simulink model "experiment_supervisor_user"  (R2025b)
settings: Solver=FixedStepDiscrete  StartTime=0.0  StopTime=inf  RelTol=1e-3
PreLoadFcn:
  | run('experiment_supervisor_data');
model workspace (MAT data in the model file):
  Ts = 0.01
undefined symbols (not defined in the file or in its folder): ControlModes, ind, MCControlModes, MCMotorParamsSet
libraries: dspswit3 x1, sldrtlib x1
settings Model: DataDictionary=amcbldc.sldd  SimulationMode=accelerator  Creator=mfussi  LastModifiedBy=rpumpo
settings OptimizationCC: GainParamInheritBuiltInType=on  DefaultUnderspecifiedDataType=single  ReuseModelBlockBuffer=off  SimCompilerOptimization=on
settings DebuggingCC: ParamSuppressDoubleToSinglePrecisionLossMsg=on  UnconnectedInputMsg=warning  UnconnectedOutputMsg=warning  UnconnectedLineMsg=warning
settings HardwareCC: ProdBitPerLong=64.0  ProdHWDeviceType=Intel->x86-64 (Linux 64)
settings ModelReferenceCC: UpdateModelReferenceTargets=IfOutOfDate  EnableRefExpFcnMdlSchedulingChecks=on
settings RTWCC: SystemTargetFile=sldrt.tlc  TemplateMakefile=sldrt.tmf  TargetLang=C++  RTWCompilerOptimization=on  GPUComputeCapability=3.5  DLArmComputeVersion=19.05  Description=Simulink Desktop Real-Time
settings CodeAppCC: MaxIdLength=95.0
settings SimulinkDesktopRealTimeCC: ExtModeTransport=0.0  ExtModeStaticAllocSize=1000000.0  TargetLibSuffix=_sldrt.a  TargetPreCompLibLocation=C:\Program Files\MATLAB\R2025b\toolbox\sldrt\lib\win64  TargetLangStandard=C++11 (ISO)  MultiwordLength=2048.0  DynamicStringBufferSize=256.0  ParMdlRefBuildCompliant=on  PreserveMATLABNamespacesInGeneratedCode=on  SubcomponentCodeInterfacePackaging=Reusable function  OptimizeReductions=on

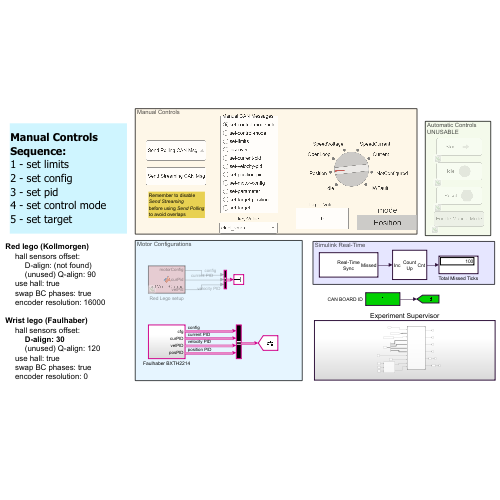
[thumbnail: Simulink's stored preview of the top-level diagram]
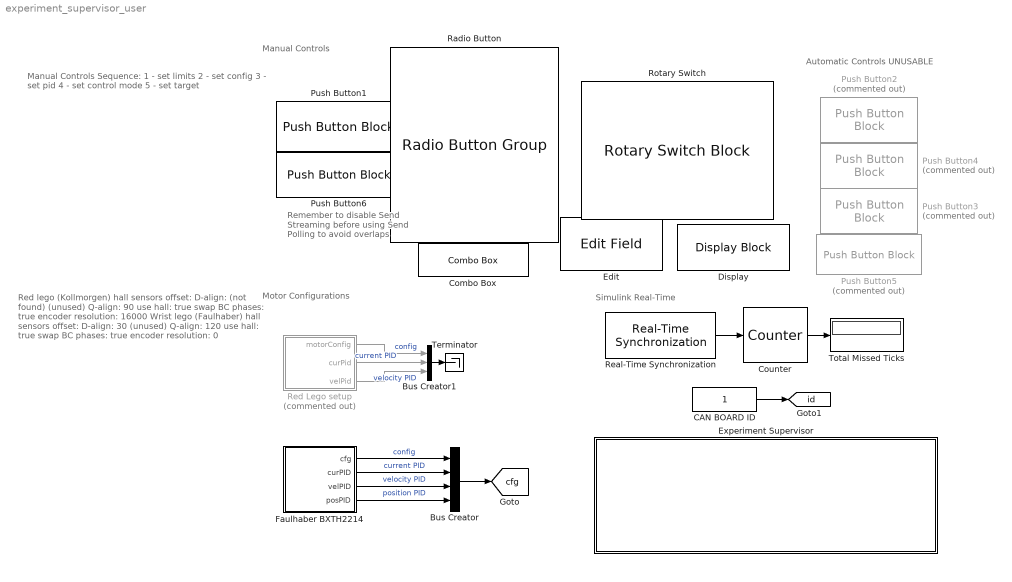
== system experiment_supervisor_user ==
  note: Manual Controls Sequence:
      | 1 - set limits
      | 2 - set config
      | 3 - set pid
      | 4 - set control mode
      | 5 - set target
  note: Motor Configurations
  note: Red lego (Kollmorgen)
      | hall sensors offset:
      | D-align: (not found)
      | (unused) Q-align: 90
      | use hall: true
      | swap BC phases: true
      | encoder resolution: 16000
      |
      | Wrist lego (Faulhaber)
      | hall sensors offset:
      | D-align: 30
      | (unused) Q-align: 120
      | use hall: true
      | swap BC phases: true
      | encoder resolution: 0
  note: Remember to disable
      | Send Streaming
      | before using Send Polling
      | to avoid overlaps
  note: Simulink Real-Time
  note: Manual Controls
  note: Automatic Controls
      | UNUSABLE
  Bus Creator : BusCreator  Inputs=4
  Bus Creator1 : BusCreator  Inputs=3
  CAN BOARD ID : Constant  OutDataTypeStr=uint32  SampleTime=0.01
  Combo Box : ComboBox  SelectedLabel=hall  UseEnumeratedDataType=on  EnumeratedDataType=MCMotorParamsSet
  Counter : dspswit3/Counter  Direction=Up  CountEvent=Rising edge  CounterSize=16 bits  MaxCount=10000  InitialCount=0  Output=Count  HitValue=32  ResetInput=off  SamplesPerFrame=1  Ts=1  CntDtype=uint16  HitDtype=Logical
  Display : DisplayBlock  Format=Integer  Transparency=1  GridColor=[0.502, 0.502, 0.502]
  Edit : EditField  ShowInitialText=on  Alignment=Center
  Experiment Supervisor : Subsystem
  Faulhaber BXTH2214 : Subsystem
  Push Button1 : PushButtonBlock  ButtonText=Send Polling CAN Msg  Icon=Triangle  IconAlignment=Right  IconOnColor=[1.0, 0.0, 1.0]  IconOffColor=[0.74901960784313726, 0.74901960784313726, 0.74901960784313726]  IconColor=On  OffValue=0.000000
  Push Button2 : PushButtonBlock  Commented=on  ButtonText=Start  Icon=TurnSignalRight  IconAlignment=Right  IconOnColor=[0.0, 1.0, 0.0]  IconOffColor=[0.74901960784313726, 0.74901960784313726, 0.74901960784313726]  IconColor=On  OffValue=-nan(ind)
  Push Button3 : PushButtonBlock  Commented=on  ButtonText=Reset  OnValue=2  Icon=Hexagon  IconAlignment=Right  IconOnColor=[1.0, 0.0, 0.0]  IconOffColor=[0.74901960784313726, 0.74901960784313726, 0.74901960784313726]  IconColor=On  OffValue=2.000000
  Push Button4 : PushButtonBlock  Commented=on  ButtonText=Idle  OnValue=0  Icon=Circle  IconAlignment=Right  IconOnColor=[1.0, 1.0, 0.0]  IconOffColor=[0.74901960784313726, 0.74901960784313726, 0.74901960784313726]  IconColor=On  OffValue=-1.000000
  Push Button5 : PushButtonBlock  Commented=on  ButtonText=Enable Manual Mode  ButtonType=Latch  IconAlignment=Right  IconOnColor=[1.0, 0.0, 1.0]  IconOffColor=[0.74901960784313726, 0.74901960784313726, 0.74901960784313726]  OffValue=0.000000
  Push Button6 : PushButtonBlock  ButtonText=Send Streaming CAN Msg  ButtonType=Latch  Icon=TurnSignalRight  IconAlignment=Right  IconOnColor=[0.0, 0.0, 1.0]  IconOffColor=[0.74901960784313726, 0.74901960784313726, 0.74901960784313726]  IconColor=On  OffValue=0.000000
  Radio Button : RadioButtonGroup  LabelPosition=Hide  SelectedLabel=set-control-mode-idle  ButtonGroupName=Manual CAN Messages
  Real-Time Synchronization : sldrtlib/Real-Time Synchronization  SampleTime=Ts  MaxMissedTicks=inf  ShowMissedTicks=on  YieldWhenWaiting=off
  Red Lego setup : MATLAB Function  Commented=on  TreatAsAtomicUnit=on
  Rotary Switch : RotarySwitchBlock  LabelPosition=Hide  UseEnumeratedDataType=on  EnumeratedDataType=MCControlModes
  Terminator : Terminator
  Total Missed Ticks : Display
      settings: Decimation=5
  tag scope: cfg=global, id=global
  wires:
  Real-Time Synchronization/1 -> Counter/1
  Faulhaber BXTH2214/1(cfg) -> Bus Creator/1  "config"
  Faulhaber BXTH2214/2(curPID) -> Bus Creator/2  "current PID"
  Faulhaber BXTH2214/3(velPID) -> Bus Creator/3  "velocity PID"
  Red Lego setup/3(velPid) -> Bus Creator1/3  "velocity PID"
  Red Lego setup/1(motorConfig) -> Bus Creator1/1  "config"
  Red Lego setup/2(curPid) -> Bus Creator1/2  "current PID"
  Bus Creator/1 -> [cfg]
  Bus Creator1/1 -> Terminator/1
  Counter/1 -> Total Missed Ticks/1
  CAN BOARD ID/1 -> [id]
  Faulhaber BXTH2214/4(posPID) -> Bus Creator/4  "position PID"

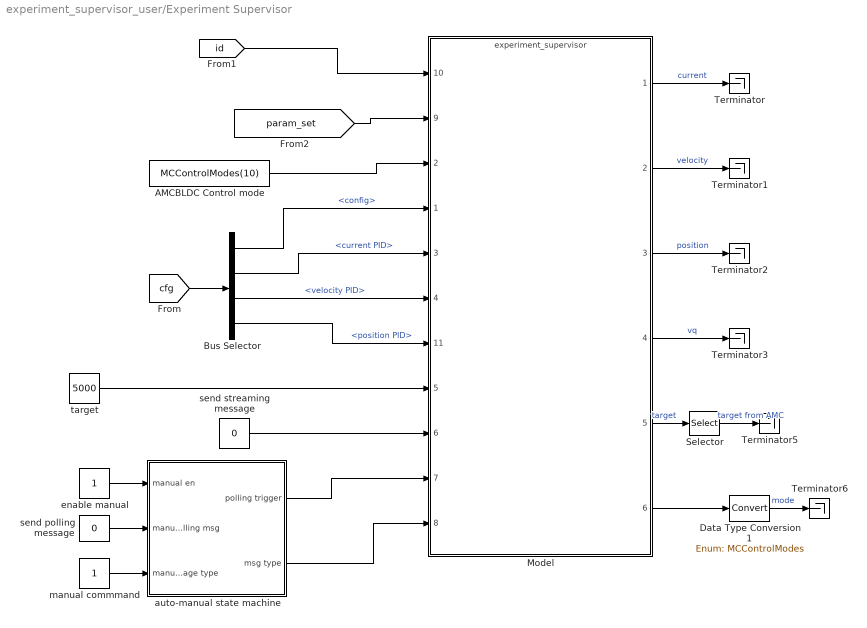
== system experiment_supervisor_user/Experiment Supervisor ==
  AMCBLDC Control mode : Constant  Value=MCControlModes(10)
  Bus Selector : BusSelector  OutputSignals=config,current PID,velocity PID,position PID
  Data Type Conversion1 : DataTypeConversion  OutDataTypeStr=Enum: MCControlModes  SaturateOnIntegerOverflow=off  RndMeth=Floor
  Model : ModelReference  ModelNameDialog=experiment_supervisor.slx  SimulationMode=Normal  ModelReferenceVersion=9.47
      settings: PortSchema="{\"entries\":[{\"content\":{\"sides\":[{\"content\":{\"connectorIds\":[\"In10\",\"In9\",\"In2\",\"In1\",\"In3\",\"In4\",\"In11\",\"In5\",\"In6\",\"In7\",\"In8\"]},\"type\":\"ConnectorPlacement.EquallySpacedRectSide\",\"uuid\":\"bfbdf898-42a5-495c-8a1e-d70d1f7414e8\"},{\"content\":{\"connectorIds\":[\"Out1\",\"Out2\",\"Out3\",\"Out4\",\"Out5\",\"Out6\"],\"side\":\"RIGHT\"},\"type\":\"ConnectorPlacement.EquallySpacedRectSide\",\"uuid\":\"3fb07422-e541-47fe-8bd2-34fc87b5d4e0\"},{\"content\":{\"side\":\"TOP\"},\"type\":\"ConnectorPlacement.EquallySpacedRectSide\",\"uuid\":\"cc070490-4dff-4736-882c-6ee4a91a824d\"}]},\"type\":\"ConnectorPlacement.EquallySpacedConnector\",\"uuid\":\"82f7e7bc-78f2-4fca-805f-7ff02feabc7a\"}],\"packageUris\":[\"http://schema.mathworks.com/mf0/Connector/R2020b\"],\"version\":\"1.0\"}"
  Selector : Selector  InputPortWidth=3  IndexOptions=Index vector (dialog)  Indices=[1]  OutputSizes=1
  Terminator{,1..3,5..6} (6 alike) : Terminator
  auto-manual state machine : Subsystem
  enable manual : Constant  OutDataTypeStr=uint8
  manual commmand : Constant  OutDataTypeStr=uint8
  send polling message : Constant  Value=0  OutDataTypeStr=uint8
  send streaming message : Constant  Value=0  OutDataTypeStr=Inherit: Inherit via back propagation
  target : Constant  Value=5000  OutDataTypeStr=single
  wires:
  Bus Selector/2 -> Model/3  "<current PID>"
  enable manual/1 -> auto-manual state machine/1(manual en)
  send polling message/1 -> auto-manual state machine/2(manual send polling msg)
  [cfg] -> Bus Selector/1
  Selector/1 -> Terminator5/1  "target from AMC"
  manual commmand/1 -> auto-manual state machine/3(manual message type)
  Model/3 -> Terminator2/1  "position"
  AMCBLDC Control mode/1 -> Model/2
  Bus Selector/1 -> Model/1  "<config>"
  Bus Selector/3 -> Model/4  "<velocity PID>"
  target/1 -> Model/5
  send streaming message/1 -> Model/6
  auto-manual state machine/1(polling trigger) -> Model/7
  Model/4 -> Terminator3/1  "vq"
  auto-manual state machine/2(msg type) -> Model/8
  Model/1 -> Terminator/1  "current"
  Model/2 -> Terminator1/1  "velocity"
  Model/5 -> Selector/1  "target"
  Model/6 -> Data Type Conversion1/1
  Data Type Conversion1/1 -> Terminator6/1  "mode"
  [id] -> Model/10
  [param_set] -> Model/9
  Bus Selector/4 -> Model/11  "<position PID>"

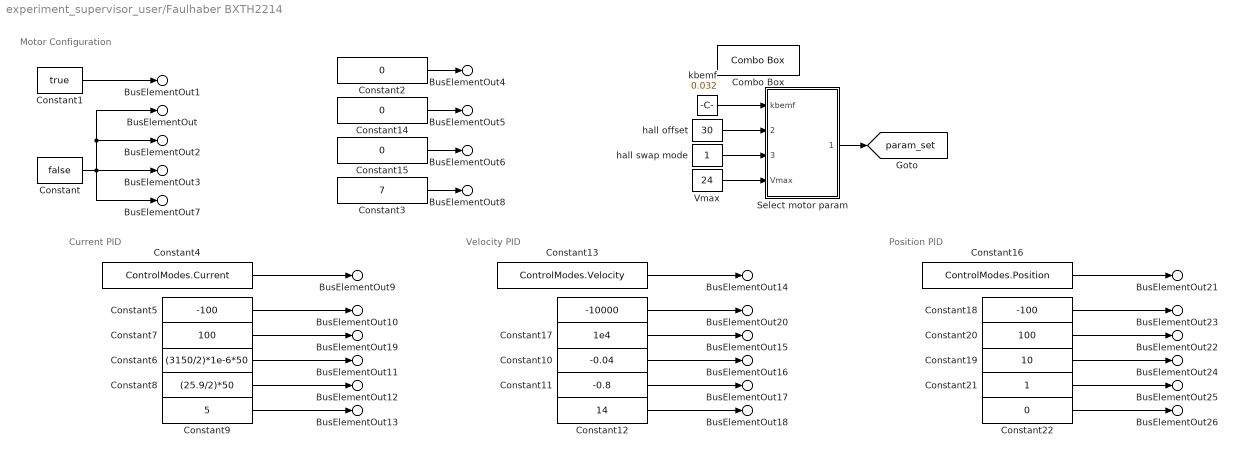
== system experiment_supervisor_user/Faulhaber BXTH2214 ==
  note: Motor Configuration
  note: Current PID
  note: Velocity PID
  note: Position PID
  " " : Constant  Value=-10000  OutDataTypeStr=Inherit: Inherit via back propagation
  Combo Box : ComboBox  SelectedLabel=hall  UseEnumeratedDataType=on  EnumeratedDataType=MCMotorParamsSet
  Constant : Constant  Value=false  OutDataTypeStr=Inherit: Inherit via back propagation
  Constant1 : Constant  Value=true  OutDataTypeStr=Inherit: Inherit via back propagation
  Constant10 : Constant  Value=-0.04  OutDataTypeStr=Inherit: Inherit via back propagation
  Constant11 : Constant  Value=-0.8  OutDataTypeStr=Inherit: Inherit via back propagation
  Constant12 : Constant  Value=14  OutDataTypeStr=Inherit: Inherit via back propagation
  Constant13 : Constant  Value=ControlModes.Velocity  OutDataTypeStr=Inherit: Inherit via back propagation
  Constant{2,14..15,22} (4 alike) : Constant  Value=0  OutDataTypeStr=Inherit: Inherit via back propagation
  Constant16 : Constant  Value=ControlModes.Position  OutDataTypeStr=Inherit: Inherit via back propagation
  Constant17 : Constant  Value=1e4  OutDataTypeStr=Inherit: Inherit via back propagation
  Constant18 : Constant  Value=-100  OutDataTypeStr=Inherit: Inherit via back propagation
  Constant19 : Constant  Value=10  OutDataTypeStr=Inherit: Inherit via back propagation
  Constant20 : Constant  Value=100  OutDataTypeStr=Inherit: Inherit via back propagation
  Constant21 : Constant  OutDataTypeStr=Inherit: Inherit via back propagation
  Constant3 : Constant  Value=7  OutDataTypeStr=Inherit: Inherit via back propagation
  Constant4 : Constant  Value=ControlModes.Current  OutDataTypeStr=Inherit: Inherit via back propagation
  Constant5 : Constant  Value=-100  OutDataTypeStr=Inherit: Inherit via back propagation
  Constant6 : Constant  Value=(3150/2)*1e-6*50  OutDataTypeStr=Inherit: Inherit via back propagation
  Constant7 : Constant  Value=100  OutDataTypeStr=Inherit: Inherit via back propagation
  Constant8 : Constant  Value=(25.9/2)*50  OutDataTypeStr=Inherit: Inherit via back propagation
  Constant9 : Constant  Value=5  OutDataTypeStr=Inherit: Inherit via back propagation
  Select motor param : Subsystem
  Vmax : Constant  Value=24  OutDataTypeStr=single
  hall offset : Constant  Value=30  OutDataTypeStr=single
  hall swap mode : Constant  OutDataTypeStr=single
  kbemf : Constant  Value=0.032  OutDataTypeStr=single
  BusElementOut : Outport  PortName=cfg  Element=enable_verbosity
  BusElementOut1 : Outport  PortName=cfg  Element=has_hall_sens
  BusElementOut2 : Outport  PortName=cfg  Element=has_quadrature_encoder
  BusElementOut3 : Outport  PortName=cfg  Element=has_temperature_sens
  BusElementOut4 : Outport  PortName=cfg  Element=encoder_tolerance
  BusElementOut8 : Outport  PortName=cfg  Element=pole_pairs
  BusElementOut5 : Outport  PortName=cfg  Element=rotor_encoder_resolution
  BusElementOut6 : Outport  PortName=cfg  Element=rotor_index_offset
  BusElementOut7 : Outport  PortName=cfg  Element=use_index
  BusElementOut9 : Outport  Port=2  PortName=curPID  Element=type
  BusElementOut19 : Outport  Port=2  PortName=curPID  Element=OutMax
  BusElementOut10 : Outport  Port=2  PortName=curPID  Element=OutMin
  BusElementOut11 : Outport  Port=2  PortName=curPID  Element=P
  BusElementOut12 : Outport  Port=2  PortName=curPID  Element=I
  BusElementOut13 : Outport  Port=2  PortName=curPID  Element=shift_factor
  BusElementOut14 : Outport  Port=3  PortName=velPID  Element=type
  BusElementOut15 : Outport  Port=3  PortName=velPID  Element=OutMax
  BusElementOut20 : Outport  Port=3  PortName=velPID  Element=OutMin
  BusElementOut16 : Outport  Port=3  PortName=velPID  Element=P
  BusElementOut17 : Outport  Port=3  PortName=velPID  Element=I
  BusElementOut18 : Outport  Port=3  PortName=velPID  Element=shift_factor
  BusElementOut21 : Outport  Port=4  PortName=posPID  Element=type
  BusElementOut22 : Outport  Port=4  PortName=posPID  Element=OutMax
  BusElementOut23 : Outport  Port=4  PortName=posPID  Element=OutMin
  BusElementOut24 : Outport  Port=4  PortName=posPID  Element=P
  BusElementOut25 : Outport  Port=4  PortName=posPID  Element=I
  BusElementOut26 : Outport  Port=4  PortName=posPID  Element=shift_factor
  tag scope: param_set=global
  wires:
  Constant/1 -> BusElementOut2/1, BusElementOut/1, BusElementOut3/1, BusElementOut7/1
  Constant1/1 -> BusElementOut1/1
  Constant2/1 -> BusElementOut4/1
  Constant3/1 -> BusElementOut8/1
  Constant4/1 -> BusElementOut9/1
  Constant5/1 -> BusElementOut10/1
  Constant6/1 -> BusElementOut11/1
  Constant7/1 -> BusElementOut19/1
  Constant8/1 -> BusElementOut12/1
  Constant9/1 -> BusElementOut13/1
  Constant11/1 -> BusElementOut17/1
  Constant12/1 -> BusElementOut18/1
  Constant10/1 -> BusElementOut16/1
  Constant13/1 -> BusElementOut14/1
  Constant14/1 -> BusElementOut5/1
  Constant15/1 -> BusElementOut6/1
  " "/1 -> BusElementOut20/1
  Constant17/1 -> BusElementOut15/1
  hall swap mode/1 -> Select motor param/3(hall swap mode)
  hall offset/1 -> Select motor param/2(hall offset)
  Vmax/1 -> Select motor param/4(Vmax)
  kbemf/1 -> Select motor param/1(kbemf)
  Select motor param/1(param_set) -> [param_set]
  Constant16/1 -> BusElementOut21/1
  Constant22/1 -> BusElementOut26/1
  Constant19/1 -> BusElementOut24/1
  Constant18/1 -> BusElementOut23/1
  Constant20/1 -> BusElementOut22/1
  Constant21/1 -> BusElementOut25/1

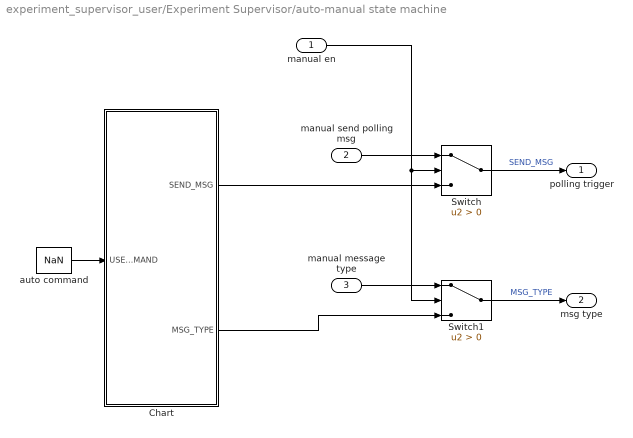
== system experiment_supervisor_user/Experiment Supervisor/auto-manual state machine ==
  manual en : Inport
  manual send polling msg : Inport  Port=2
  manual message type : Inport  Port=3
  Chart : Stateflow chart  TreatAsAtomicUnit=on
      settings: PortSchema="{\"entries\":[{\"content\":{\"sides\":[{\"content\":{\"connectorIds\":[\"In1\"]},\"type\":\"ConnectorPlacement.EquallySpacedRectSide\",\"uuid\":\"3f3ecf7a-eca8-49e2-a594-4c8df01bcae2\"},{\"content\":{\"connectorIds\":[\"Out2\",\"Out1\"],\"side\":\"RIGHT\"},\"type\":\"ConnectorPlacement.EquallySpacedRectSide\",\"uuid\":\"2e405059-6050-4daf-b42b-e1c8d6f3a572\"},{\"content\":{\"side\":\"TOP\"},\"type\":\"ConnectorPlacement.EquallySpacedRectSide\",\"uuid\":\"8705f6e5-e301-4990-b24d-44270950b42f\"}]},\"type\":\"ConnectorPlacement.EquallySpacedConnector\",\"uuid\":\"46b9b7aa-14e0-48f8-b8fe-455c7835f2bb\"}],\"packageUris\":[\"http://schema.mathworks.com/mf0/Connector/R2020b\"],\"version\":\"1.0\"}"
  Switch : Switch  Criteria=u2 > Threshold  SaturateOnIntegerOverflow=off  InputSameDT=off
  Switch1 : Switch  Criteria=u2 > Threshold  SaturateOnIntegerOverflow=off  InputSameDT=off
  auto command : Constant  Value=NaN
  polling trigger : Outport
  msg type : Outport  Port=2
  wires:
  manual en/1 -> Switch1/2, Switch/2
  manual message type/1 -> Switch1/1
  Chart/2(SEND_MSG) -> Switch/3
  Chart/1(MSG_TYPE) -> Switch1/3
  auto command/1 -> Chart/1(USER_COMMAND)
  manual send polling msg/1 -> Switch/1
  Switch1/1 -> msg type/1  "MSG_TYPE"
  Switch/1 -> polling trigger/1  "SEND_MSG"

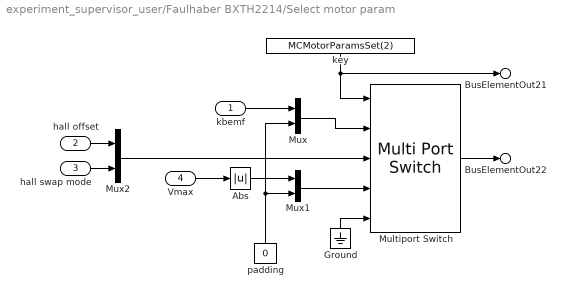
== system experiment_supervisor_user/Faulhaber BXTH2214/Select motor param ==
  kbemf : Inport
  hall offset : Inport  Port=2
  hall swap mode : Inport  Port=3
  Vmax : Inport  Port=4  OutDataTypeStr=single
  Abs : Abs  SaturateOnIntegerOverflow=off
  Ground : Ground
  Multiport Switch : MultiPortSwitch  DataPortOrder=Specify indices  DataPortIndices={MCMotorParamsSet.Kbemf, MCMotorParamsSet.hall, MCMotorParamsSet.elect_vmax}  DataPortForDefault=Additional data port  DiagnosticForDefault=None  SaturateOnIntegerOverflow=off  InputSameDT=off
  Mux : Mux  Inputs=2
  Mux1 : Mux  Inputs=2
  Mux2 : Mux  Inputs=2
  key : Constant  Value=MCMotorParamsSet(2)  OutDataTypeStr=Enum: MCMotorParamsSet
  padding : Constant  Value=0  OutDataTypeStr=single
  BusElementOut21 : Outport  PortName=param_set  Element=key
  BusElementOut22 : Outport  PortName=param_set  Element=value
  wires:
  Mux/1 -> Multiport Switch/2
  kbemf/1 -> Mux/1
  Mux2/1 -> Multiport Switch/3
  Mux1/1 -> Multiport Switch/4
  Ground/1 -> Multiport Switch/5
  padding/1 -> Mux/2, Mux1/2
  hall offset/1 -> Mux2/1
  hall swap mode/1 -> Mux2/2
  Vmax/1 -> Abs/1
  key/1 -> BusElementOut21/1, Multiport Switch/1
  Multiport Switch/1 -> BusElementOut22/1
  Abs/1 -> Mux1/1

== stateflow chart experiment_supervisor_user/Experiment Supervisor/auto-manual state machine/Chart ==
  state RESET_IDLE
    entry:
    SEND_MSG=1;
    on after(1, sec):
    SEND_MSG=0;
  state WAIT_LIMITS
    entry:
    SEND_MSG=1;
    on after(1, sec):
    SEND_MSG=0;
  state IDLE
    entry:
    SEND_MSG=1;
    on after(1 , sec):
    SEND_MSG=0;
  state STARTED
    entry:
    SEND_MSG=1;
    on after(1 , sec):
    SEND_MSG=0;
  state WAIT_CTRL_MODE
    entry:
    SEND_MSG=1;
    on after(1,sec):
    SEND_MSG=0;
  (default) -> RESET_IDLE
  STARTED -> RESET_IDLE [order 3] : [USER_COMMAND == 2]
      | {MSG_TYPE = 1;}
  RESET_IDLE -> WAIT_LIMITS [order 1] : [USER_COMMAND == 1]
      | {MSG_TYPE = 4;}
  IDLE -> RESET_IDLE [order 2] : [USER_COMMAND == 2]
      | {MSG_TYPE=1;}
  WAIT_LIMITS -> RESET_IDLE [order 2] : [USER_COMMAND == 2]
      | {MSG_TYPE = 1;}
  RESET_IDLE -> RESET_IDLE [order 2] : [USER_COMMAND == 2]
      | {MSG_TYPE=1;}
  WAIT_CTRL_MODE -> RESET_IDLE [order 2] : [USER_COMMAND == 2]
      | {MSG_TYPE = 1;}
  IDLE -> IDLE [order 3] : [USER_COMMAND == 0 ]
      | {MSG_TYPE=1;}
  WAIT_LIMITS -> WAIT_CTRL_MODE [order 1] : after(2, sec){MSG_TYPE = 2;}
  STARTED -> IDLE [order 1] : [USER_COMMAND == 0 ]
      | {MSG_TYPE=1;}
  IDLE -> WAIT_CTRL_MODE [order 1] : [USER_COMMAND == 1]
      | {MSG_TYPE = 2;}
  WAIT_CTRL_MODE -> STARTED [order 1] : after(2, sec){MSG_TYPE=3;}
  STARTED -> STARTED [order 2] : [USER_COMMAND == 1]{MSG_TYPE = 3;}
  data: MSG_TYPE output uint8 =uint8(1); USER_COMMAND input; SEND_MSG output uint8 =uint8(0)

== matlab function experiment_supervisor_user/Red Lego setup ==
  data: motorConfig output Bus: MotorConfig; curPid output Bus: PIDConfig; velPid output Bus: PIDConfig
function [motorConfig, curPid, velPid] = setMotorConfig()

motorConfig.hall_sens_offset = single(30); % deg
motorConfig.has_hall_sens = true;
motorConfig.has_quadrature_encoder = true;
motorConfig.has_speed_quadrature_encoder = false;
motorConfig.has_torque_sens = false;
motorConfig.use_index = false;
motorConfig.enable_verbosity = true;
motorConfig.rotor_encoder_resolution = int16(16000);
motorConfig.rotor_index_offset = int16(0);
motorConfig.encoder_tolerance = uint8(0);
motorConfig.pole_pairs = uint8(4);
motorConfig.Kbemf = single(0);
motorConfig.Rphase = single(0);
motorConfig.Imin = single(-1e3);
motorConfig.Imax = single(1e3);
motorConfig.Vcc = single(24);
motorConfig.Vmax = single(24);

% Hall offset and BC phases swap is not available as a CAN message
% The parameters need to be changed in rtw_motor_config.c
swap_bc = 1;

% ---------------------------------

curPid.OutMax = single(100);
curPid.OutMin = single(-100);
curPid.P = single(2);
curPid.I = single(500);
curPid.D = single(0);
curPid.N = single(100);
curPid.I0 = single(0);
curPid.D0 = single(0);
curPid.shift_factor = uint8(0);


velPid.OutMax = single(1000);
velPid.OutMin = single(-1000);
velPid.P = single(1000);
velPid.I = single(1000);
velPid.D = single(0);
velPid.N = single(100);
velPid.I0 = single(0);
velPid.D0 = single(0);
velPid.shift_factor = uint8(10);
